simulink model "ball_balancing_omni3_multibody_lqi_rev1_r2024b"  (R2024b)
settings: Solver=VariableStepAuto  StartTime=0.0  StopTime=50  MaxStep=1e-3  MinStep=1e-6  RelTol=ballbotParams.simulation.relativeTolerance
PreLoadFcn:
  | if ~exist('ballbotParams','var'), ballbotParams = ballbotRev1Parameters; end
InitFcn:
  | if ~exist('ballbotParams','var') || ~isfield(ballbotParams,'parameterSource') || ballbotParams.parameterSource ~= "ballbotRev1Parameters" || ~isfield(ballbotParams,'controller') || ~isfield(ballbotParams,'estimator') || ~isfield(ballbotParams.controller,'torqueDrive') || ~isfield(ballbotParams.controller.torqueDrive,'propulsionGain') || ~isfield(ballbotParams.estimator,'truthDelaySteps') || ~isfield(ballbotParams.controller.torqueLqi,'robustness'), ballbotParams = ballbotRev1Parameters; end
  | % ballbotRev1RuntimeApply: re-apply runtime solver/driver/plant settings on every sim start.
  | clear functions;
  | ballbotRev1SimConfig;
  | if exist('ballbotParams','var'), ballbotRev1PlantAugment(bdroot, ballbotParams); end
values from neighbouring files (symbols this model uses):
  N = 0    [ballbotRollingResistance.m]
  s = result.spec    [ballbotBenchmark.m]
undefined symbols (not defined in the file or in its folder): ballbotCustomFriction, ballbotEstimatorInitialState, ballbotEstimatorUpdate, ballbotEulerToQuaternion, ballbotImuFromJoint, ballbotLqiControllerUpdate, ballbotLqiFeedbackState, ballbotMdd3aGateDrive, ballbotParams, ballbotPoseFromJoint, ballbotRev1CommandProfile, ballbotRollingResistance, ballbotRoverInitialPosition, ballbotShaftFrictionTorque, ballbotTorqueDutyStep, ballbotTruthGate, ballbotWheelRateFromDisplacement, X, Y, Z
libraries: nesl_utility x54, sm_lib x28, fl_lib x21, ee_lib x6
(part 2 of 3)

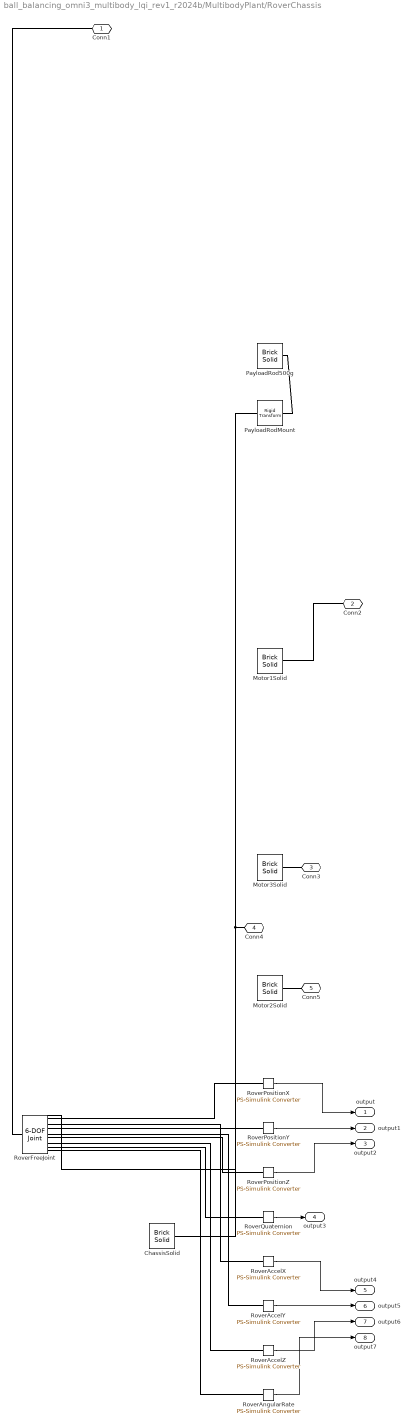
== system ball_balancing_omni3_multibody_lqi_rev1_r2024b/MultibodyPlant/RoverChassis ==
  ChassisSolid : sm_lib/Body Elements/Brick Solid  BrickDimensions=[0.12 0.12 ballbotParams.rover.chassisHeight]  BrickDimensionsUnits=m  ExportEntireGeometry=off  InertiaType=Custom  BasedOnType=Mass  Density=1000  DensityUnits=kg/m^3  Mass=ballbotParams.rover.bodyMass  MassUnits=kg  CenterOfMass=[0 0 ballbotParams.rover.bodyComAboveBall - ballbotParams.rover.centerAboveBall]  CenterOfMassUnits=m  MomentsOfInertia=ballbotParams.rover.bodyInertia.'  MomentsOfInertiaUnits=kg*m^2  ProductsOfInertia=[0 0 0]  ProductsOfInertiaUnits=kg*m^2  GraphicType=FromGeometry  MarkerShape=Sphere  MarkerSize=10  GraphicVisPropType=SimpleVisualProperties  GraphicDiffuseColor=[0.85 0.25 0.10 1.0]  GraphicOpacity=1  GraphicSpecularColor=[0.5 0.5 0.5 1.0]  GraphicAmbientColor=[0.15 0.15 0.15 1.0]  GraphicEmissiveColor=[0.0 0.0 0.0 1.0]  GraphicShininess=75  DoExposeReferenceFrame=on  SerializedFrames=<Frames/>
  Motor1Solid : sm_lib/Body Elements/Brick Solid  BrickDimensions=ballbotParams.motor.dimensions  BrickDimensionsUnits=m  ExportEntireGeometry=off  InertiaType=CalculateFromGeometry  BasedOnType=Mass  Density=1000  DensityUnits=kg/m^3  Mass=ballbotParams.motor.mass  MassUnits=kg  CenterOfMass=[0 0 0]  CenterOfMassUnits=m  MomentsOfInertia=[1 1 1]  MomentsOfInertiaUnits=kg*m^2  ProductsOfInertia=[0 0 0]  ProductsOfInertiaUnits=kg*m^2  GraphicType=FromGeometry  MarkerShape=Sphere  MarkerSize=10  GraphicVisPropType=SimpleVisualProperties  GraphicDiffuseColor=[0.25 0.25 0.25 1.0]  GraphicOpacity=1  GraphicSpecularColor=[0.5 0.5 0.5 1.0]  GraphicAmbientColor=[0.15 0.15 0.15 1.0]  GraphicEmissiveColor=[0.0 0.0 0.0 1.0]  GraphicShininess=75  DoExposeReferenceFrame=on  SerializedFrames=<Frames/>
  Motor2Solid : sm_lib/Body Elements/Brick Solid  BrickDimensions=ballbotParams.motor.dimensions  BrickDimensionsUnits=m  ExportEntireGeometry=off  InertiaType=CalculateFromGeometry  BasedOnType=Mass  Density=1000  DensityUnits=kg/m^3  Mass=ballbotParams.motor.mass  MassUnits=kg  CenterOfMass=[0 0 0]  CenterOfMassUnits=m  MomentsOfInertia=[1 1 1]  MomentsOfInertiaUnits=kg*m^2  ProductsOfInertia=[0 0 0]  ProductsOfInertiaUnits=kg*m^2  GraphicType=FromGeometry  MarkerShape=Sphere  MarkerSize=10  GraphicVisPropType=SimpleVisualProperties  GraphicDiffuseColor=[0.5 0.5 0.5]  GraphicOpacity=1  GraphicSpecularColor=[0.5 0.5 0.5 1.0]  GraphicAmbientColor=[0.15 0.15 0.15 1.0]  GraphicEmissiveColor=[0.0 0.0 0.0 1.0]  GraphicShininess=75  DoExposeReferenceFrame=on  SerializedFrames=<Frames/>
  Motor3Solid : sm_lib/Body Elements/Brick Solid  BrickDimensions=ballbotParams.motor.dimensions  BrickDimensionsUnits=m  ExportEntireGeometry=off  InertiaType=CalculateFromGeometry  BasedOnType=Mass  Density=1000  DensityUnits=kg/m^3  Mass=ballbotParams.motor.mass  MassUnits=kg  CenterOfMass=[0 0 0]  CenterOfMassUnits=m  MomentsOfInertia=[1 1 1]  MomentsOfInertiaUnits=kg*m^2  ProductsOfInertia=[0 0 0]  ProductsOfInertiaUnits=kg*m^2  GraphicType=FromGeometry  MarkerShape=Sphere  MarkerSize=10  GraphicVisPropType=SimpleVisualProperties  GraphicDiffuseColor=[0.5 0.5 0.5]  GraphicOpacity=1  GraphicSpecularColor=[0.5 0.5 0.5 1.0]  GraphicAmbientColor=[0.15 0.15 0.15 1.0]  GraphicEmissiveColor=[0.0 0.0 0.0 1.0]  GraphicShininess=75  DoExposeReferenceFrame=on  SerializedFrames=<Frames/>
  PayloadRod500g : sm_lib/Body Elements/Brick Solid  BrickDimensions=[ballbotParams.fullplant.payload.width ballbotParams.fullplant.payload.width ballbotParams.fullplant.payload.length]  BrickDimensionsUnits=m  ExportEntireGeometry=off  InertiaType=CalculateFromGeometry  BasedOnType=Density  Density=1000  DensityUnits=kg/m^3  Mass=ballbotParams.fullplant.payload.mass  MassUnits=kg  CenterOfMass=[0 0 0]  CenterOfMassUnits=m  MomentsOfInertia=[1 1 1]  MomentsOfInertiaUnits=kg*m^2  ProductsOfInertia=[0 0 0]  ProductsOfInertiaUnits=kg*m^2  GraphicType=FromGeometry  MarkerShape=Sphere  MarkerSize=10  GraphicVisPropType=SimpleVisualProperties  GraphicDiffuseColor=[0.5 0.5 0.5]  GraphicOpacity=1  GraphicSpecularColor=[0.5 0.5 0.5 1.0]  GraphicAmbientColor=[0.15 0.15 0.15 1.0]  GraphicEmissiveColor=[0.0 0.0 0.0 1.0]  GraphicShininess=75  DoExposeReferenceFrame=on  SerializedFrames=<Frames/>
  PayloadRodMount : sm_lib/Frames and Transforms/Rigid Transform  RotationMethod=None  FollAlignAxisA=+X  BaseAlignAxisA=+Y  FollAlignAxisB=+Y  BaseAlignAxisB=+Z  RotationStandardAxis=+Z  RotationAngle=0  RotationAngleUnits=deg  RotationArbitraryAxis=[0 0 1]  RotationSequenceAxes=FollowerAxes  RotationSequence=XYX  RotationSequenceAngles=[0 0 0]  RotationSequenceAnglesUnits=deg  RotationMatrix=[1 0 0;0 1 0;0 0 1]  Quaternion=[1 0 0 0]  TranslationMethod=Cartesian  TranslationCartesianOffset=[0 0 0.165]  TranslationCartesianOffsetUnits=m  TranslationStandardAxis=+Z  TranslationStandardOffset=0  TranslationStandardOffsetUnits=m  TranslationROffset=0  TranslationROffsetUnits=m  TranslationThetaOffset=0  TranslationThetaOffsetUnits=deg  TranslationZOffset=0  TranslationZOffsetUnits=m
  RoverAccelX : nesl_utility/PS-Simulink Converter  PhysicalDomain=network_engine_domain  SubClassName=ps_output  LeftPortType=input  RightPortType=output  PseudoPeriodic=off  Frequencies=[]  VectorFormat=inherit  Unit=m/s^2  AffineConversion=off
  RoverAccelY : nesl_utility/PS-Simulink Converter  PhysicalDomain=network_engine_domain  SubClassName=ps_output  LeftPortType=input  RightPortType=output  PseudoPeriodic=off  Frequencies=[]  VectorFormat=inherit  Unit=m/s^2  AffineConversion=off
  RoverAccelZ : nesl_utility/PS-Simulink Converter  PhysicalDomain=network_engine_domain  SubClassName=ps_output  LeftPortType=input  RightPortType=output  PseudoPeriodic=off  Frequencies=[]  VectorFormat=inherit  Unit=m/s^2  AffineConversion=off
  RoverAngularRate : nesl_utility/PS-Simulink Converter  PhysicalDomain=network_engine_domain  SubClassName=ps_output  LeftPortType=input  RightPortType=output  PseudoPeriodic=off  Frequencies=[]  VectorFormat=inherit  Unit=rad/s  AffineConversion=off
  RoverFreeJoint : sm_lib/Joints/6-DOF Joint  JointMode=Normal  CompositeWrenchDir=FollowerOnBase  CompositeWrenchFrame=BaseFrame  SenseConstraintForce=off  SenseConstraintTorque=off  SenseTotalForce=off  SenseTotalTorque=off  PxPositionTargetSpecify=on  PxPositionTargetPriority=High  PxPositionTargetValue=ballbotRoverInitialPosition(ballbotParams,1)  PxPositionTargetValueUnits=m  PxVelocityTargetSpecify=off  PxVelocityTargetPriority=High  PxVelocityTargetValue=0  PxVelocityTargetValueUnits=m/s  PxEquilibriumPosition=0  PxEquilibriumPositionUnits=m  PxSpringStiffness=0  PxSpringStiffnessUnits=N/m  PxDampingCoefficient=0  PxDampingCoefficientUnits=N/(m/s)  PxLowerLimitSpecify=off  PxLowerLimitBound=-1  PxLowerLimitBoundUnits=m  PxLowerLimitStiffness=1e6  PxLowerLimitStiffnessUnits=N/m  PxLowerLimitDamping=1e3  PxLowerLimitDampingUnits=N/(m/s)  PxLowerLimitTransitionRegionWidth=1e-4  PxLowerLimitTransitionRegionWidthUnits=m  PxUpperLimitSpecify=off  PxUpperLimitBound=1  PxUpperLimitBoundUnits=m  PxUpperLimitStiffness=1e6  PxUpperLimitStiffnessUnits=N/m  PxUpperLimitDamping=1e3  PxUpperLimitDampingUnits=N/(m/s)  PxUpperLimitTransitionRegionWidth=1e-4  PxUpperLimitTransitionRegionWidthUnits=m  PxTorqueActuationMode=NoTorque  PxMotionActuationMode=ComputedMotion  PxSensePosition=on  PxSenseVelocity=on  PxSenseAcceleration=on  PxSenseTorqueForce=off  PxSenseLowerLimitTorqueForce=off  PxSenseUpperLimitTorqueForce=off  PyPositionTargetSpecify=on  PyPositionTargetPriority=High  PyPositionTargetValue=ballbotRoverInitialPosition(ballbotParams,2)  PyPositionTargetValueUnits=m  PyVelocityTargetSpecify=off  PyVelocityTargetPriority=High  PyVelocityTargetValue=0  PyVelocityTargetValueUnits=m/s  PyEquilibriumPosition=0  PyEquilibriumPositionUnits=m  PySpringStiffness=0  PySpringStiffnessUnits=N/m  PyDampingCoefficient=0  PyDampingCoefficientUnits=N/(m/s)  PyLowerLimitSpecify=off  PyLowerLimitBound=-1  PyLowerLimitBoundUnits=m  PyLowerLimitStiffness=1e6  PyLowerLimitStiffnessUnits=N/m  PyLowerLimitDamping=1e3  PyLowerLimitDampingUnits=N/(m/s)  PyLowerLimitTransitionRegionWidth=1e-4  PyLowerLimitTransitionRegionWidthUnits=m  PyUpperLimitSpecify=off  PyUpperLimitBound=1  PyUpperLimitBoundUnits=m  PyUpperLimitStiffness=1e6  PyUpperLimitStiffnessUnits=N/m  PyUpperLimitDamping=1e3  PyUpperLimitDampingUnits=N/(m/s)  PyUpperLimitTransitionRegionWidth=1e-4  PyUpperLimitTransitionRegionWidthUnits=m  PyTorqueActuationMode=NoTorque  PyMotionActuationMode=ComputedMotion  PySensePosition=on  PySenseVelocity=on  PySenseAcceleration=on  PySenseTorqueForce=off  PySenseLowerLimitTorqueForce=off  PySenseUpperLimitTorqueForce=off  PzPositionTargetSpecify=on  PzPositionTargetPriority=High  PzPositionTargetValue=ballbotRoverInitialPosition(ballbotParams,3)  PzPositionTargetValueUnits=m  PzVelocityTargetSpecify=off  PzVelocityTargetPriority=High  PzVelocityTargetValue=0  PzVelocityTargetValueUnits=m/s  PzEquilibriumPosition=0  PzEquilibriumPositionUnits=m  PzSpringStiffness=0  PzSpringStiffnessUnits=N/m  PzDampingCoefficient=0  PzDampingCoefficientUnits=N/(m/s)  PzLowerLimitSpecify=off  PzLowerLimitBound=-1  PzLowerLimitBoundUnits=m  PzLowerLimitStiffness=1e6  PzLowerLimitStiffnessUnits=N/m  PzLowerLimitDamping=1e3  PzLowerLimitDampingUnits=N/(m/s)  PzLowerLimitTransitionRegionWidth=1e-4  PzLowerLimitTransitionRegionWidthUnits=m  PzUpperLimitSpecify=off  PzUpperLimitBound=1  PzUpperLimitBoundUnits=m  PzUpperLimitStiffness=1e6  PzUpperLimitStiffnessUnits=N/m  PzUpperLimitDamping=1e3  PzUpperLimitDampingUnits=N/(m/s)  PzUpperLimitTransitionRegionWidth=1e-4  PzUpperLimitTransitionRegionWidthUnits=m  PzTorqueActuationMode=NoTorque  PzMotionActuationMode=ComputedMotion  PzSensePosition=on  PzSenseVelocity=on  PzSenseAcceleration=on  PzSenseTorqueForce=off  PzSenseLowerLimitTorqueForce=off  PzSenseUpperLimitTorqueForce=off  SphPositionTargetSpecify=on  SphPositionTargetPriority=High  SphPositionTargetRotationMethod=Quaternion  SphPositionTargetFollAlignAxisA=+X  SphPositionTargetBaseAlignAxisA=+Y  SphPositionTargetFollAlignAxisB=+Y  SphPositionTargetBaseAlignAxisB=+Z  SphPositionTargetRotationStandardAxis=+Z  SphPositionTargetRotationAngle=0  SphPositionTargetRotationAngleUnits=deg  SphPositionTargetRotationArbitraryAxis=[0 0 1]  SphPositionTargetRotationSequenceAxes=FollowerAxes  SphPositionTargetRotationSequence=XYX  SphPositionTargetRotationSequenceAngles=[0 0 0]  SphPositionTargetRotationSequenceAnglesUnits=deg  SphPositionTargetRotationMatrix=[1 0 0;0 1 0;0 0 1]  SphPositionTargetQuaternion=ballbotEulerToQuaternion(ballbotParams.rover.initialEulerWorld)  SphVelocityTargetSpecify=off  SphVelocityTargetPriority=High  SphVelocityTargetValue=[0 0 0]  SphVelocityTargetValueUnits=deg/s  SphVelocityTargetInFollowerFrame=on  SphEqPosRotationMethod=None  SphEqPosFollAlignAxisA=+X  SphEqPosBaseAlignAxisA=+Y  SphEqPosFollAlignAxisB=+Y  SphEqPosBaseAlignAxisB=+Z  SphEqPosRotationStandardAxis=+Z  SphEqPosRotationAngle=0  SphEqPosRotationAngleUnits=deg  SphEqPosRotationArbitraryAxis=[0 0 1]  SphEqPosRotationSequenceAxes=FollowerAxes  SphEqPosRotationSequence=XYX  SphEqPosRotationSequenceAngles=[0 0 0]  SphEqPosRotationSequenceAnglesUnits=deg  SphEqPosRotationMatrix=[1 0 0;0 1 0;0 0 1]  SphEqPosQuaternion=[1 0 0 0]  SphSpringStiffness=0  SphSpringStiffnessUnits=N*m/deg  SphDampingCoefficient=0  SphDampingCoefficientUnits=N*m/(deg/s)  SphLowerLimitSpecify=off  SphLowerLimitBound=15  SphLowerLimitBoundUnits=deg  SphLowerLimitStiffness=1e4  SphLowerLimitStiffnessUnits=N*m/deg  SphLowerLimitDamping=10  SphLowerLimitDampingUnits=N*m/(deg/s)  SphLowerLimitTransitionRegionWidth=0.1  SphLowerLimitTransitionRegionWidthUnits=deg  SphUpperLimitSpecify=off  SphUpperLimitBound=45  SphUpperLimitBoundUnits=deg  SphUpperLimitStiffness=1e4  SphUpperLimitStiffnessUnits=N*m/deg  SphUpperLimitDamping=10  SphUpperLimitDampingUnits=N*m/(deg/s)  SphUpperLimitTransitionRegionWidth=0.1  SphUpperLimitTransitionRegionWidthUnits=deg  SphTorqueActuationMode=NoTorque  SphActuateTorqueX=off  SphActuateTorqueY=off  SphActuateTorqueZ=off  SphActuateTorque=off  SphActuationFrame=BaseFrame  SphSensePosition=on  SphSenseVelocityX=off  SphSenseVelocityY=off  SphSenseVelocityZ=off  SphSenseVelocity=on  SphSenseAccelerationX=off  SphSenseAccelerationY=off  SphSenseAccelerationZ=off  SphSenseAcceleration=on  SphSenseLowerLimitTorqueMag=off  SphSenseUpperLimitTorqueMag=off  SphSensingFrame=BaseFrame
  RoverPositionX : nesl_utility/PS-Simulink Converter  PhysicalDomain=network_engine_domain  SubClassName=ps_output  LeftPortType=input  RightPortType=output  PseudoPeriodic=off  Frequencies=[]  VectorFormat=inherit  Unit=m  AffineConversion=off
  RoverPositionY : nesl_utility/PS-Simulink Converter  PhysicalDomain=network_engine_domain  SubClassName=ps_output  LeftPortType=input  RightPortType=output  PseudoPeriodic=off  Frequencies=[]  VectorFormat=inherit  Unit=m  AffineConversion=off
  RoverPositionZ : nesl_utility/PS-Simulink Converter  PhysicalDomain=network_engine_domain  SubClassName=ps_output  LeftPortType=input  RightPortType=output  PseudoPeriodic=off  Frequencies=[]  VectorFormat=inherit  Unit=m  AffineConversion=off
  RoverQuaternion : nesl_utility/PS-Simulink Converter  PhysicalDomain=network_engine_domain  SubClassName=ps_output  LeftPortType=input  RightPortType=output  PseudoPeriodic=off  Frequencies=[]  VectorFormat=inherit  Unit=1  AffineConversion=off
  Conn1 : PMIOPort  Side=Left
  Conn2 : PMIOPort  Port=2  Side=Right
  Conn3 : PMIOPort  Port=3  Side=Right
  Conn4 : PMIOPort  Port=4  Side=Right
  Conn5 : PMIOPort  Port=5  Side=Right
  output : Outport
  output1 : Outport  Port=2
  output2 : Outport  Port=3
  output3 : Outport  Port=4
  output4 : Outport  Port=5
  output5 : Outport  Port=6
  output6 : Outport  Port=7
  output7 : Outport  Port=8
  wires:
  RoverAccelX/1 -> output4/1
  RoverPositionY/1 -> output1/1
  RoverAngularRate/1 -> output7/1
  RoverPositionX/1 -> output/1
  RoverAccelY/1 -> output5/1
  RoverPositionZ/1 -> output2/1
  RoverAccelZ/1 -> output6/1
  RoverQuaternion/1 -> output3/1
  connections:
  RoverFreeJoint/RConn4 -- RoverAccelX/LConn1
  RoverFreeJoint/RConn2 -- RoverPositionX/LConn1
  RoverFreeJoint/RConn11 -- RoverQuaternion/LConn1
  Conn3/RConn1 -- Motor3Solid/RConn1
  Conn2/RConn1 -- Motor1Solid/RConn1
  PayloadRodMount/RConn1 -- PayloadRod500g/RConn1
  RoverFreeJoint/RConn8 -- RoverPositionZ/LConn1
  RoverFreeJoint/RConn7 -- RoverAccelY/LConn1
  RoverFreeJoint/RConn10 -- RoverAccelZ/LConn1
  RoverFreeJoint/RConn12 -- RoverAngularRate/LConn1
  Conn5/RConn1 -- Motor2Solid/RConn1
  RoverFreeJoint/RConn5 -- RoverPositionY/LConn1
  Conn1/RConn1 -- RoverFreeJoint/LConn1
  Conn4/RConn1 -- RoverFreeJoint/RConn1 -- ChassisSolid/RConn1 -- PayloadRodMount/LConn1

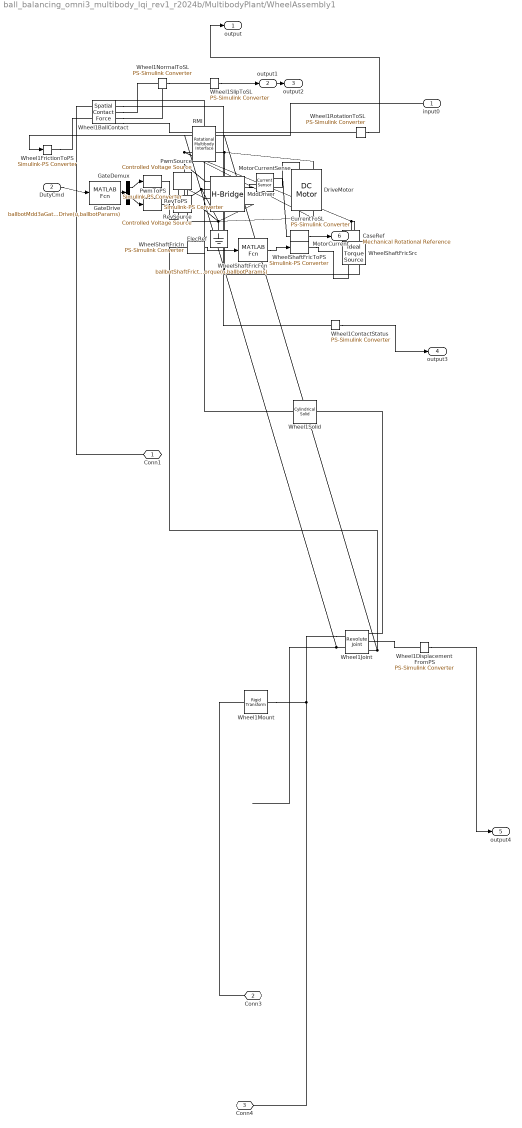
== system ball_balancing_omni3_multibody_lqi_rev1_r2024b/MultibodyPlant/WheelAssembly1 ==
  input0 : Inport
  DutyCmd : Inport  Port=2
  CaseRef : fl_lib/Mechanical/Rotational Elements/Mechanical Rotational Reference
  CurrentToSL : nesl_utility/PS-Simulink Converter  PhysicalDomain=network_engine_domain  SubClassName=ps_output  LeftPortType=input  RightPortType=output  PseudoPeriodic=off  Frequencies=[]  VectorFormat=inherit  Unit=A  AffineConversion=off
  DriveMotor : ee_lib/Electromechanical/Brushed Motors/DC Motor  field_option=ee.enum.field_option.pm  Rf=100 Ohm  Lf=1 H  Laf=0.15 H  If0=0 A  parameterization=ee.enum.dcparam_option.circuit_param  Ra=ballbotParams.motor.armatureResistance Ohm  La=ballbotParams.motor.armatureInductance H  emf_or_torque=ee.enum.emf_or_torque.ki  Kv=0.072e-3 V/rpm  Ki=ballbotParams.motor.torqueConstant N*m/A  T_stall=0.24e-3 N*m  w_max=19100 rpm  w_rated=15000 rpm  P_rated=0.08 W  V_rated=1.5 V  lam_param=ee.enum.lam_param.damping  i_noload=0 A  V_i_noload=1.5 V  J=ballbotParams.motor.equivalentInertia kg*m^2  lam=ballbotParams.motor.viscousFriction*ballbotParams.motor.viscousShare N*m*s/rad  speed0=0 rpm  alpha=3.93e-3 1/K  Tmeas=25 degC  thermal_mass=100 J/K  initial_temperature=25 degC
  ElecRef : fl_lib/Electrical/Electrical Elements/Electrical Reference
  GateDemux : Demux  Outputs=2
  GateDrive : MATLABFcn  MATLABFcn=ballbotMdd3aGateDrive(u,ballbotParams)  OutputDimensions=2
  MddDriver : ee_lib/Semiconductors & Converters/Converters/H-Bridge  pwm_or_av=ee.enum.pwm_or_av.averaged  discontinuous=ee.enum.current_profile.continuous  freewheeling_mode=ee.enum.converters.freewheeling_mode.one_switch_one_diode  Rload=10 Ohm  Lload=1e-5 H  F=ballbotParams.driver.pwmFrequency Hz  supply_ports=ee.enum.supply_ports.hidesupply  regenerative_braking_mode=ee.enum.converters.regenerative_braking_mode.always_enabled  Venable=ballbotParams.driver.enableThresholdVoltage V  Vmax=ballbotParams.driver.logicHighVoltage V  Vreverse=ballbotParams.driver.reverseThresholdVoltage V  Vbrake=ballbotParams.driver.brakeThresholdVoltage V  Vm=ballbotParams.driver.supplyVoltage V  Ron=ballbotParams.driver.bridgeOnResistance Ohm  Don=0.05 Ohm  Goff=1e-6 S  Tmeas=298.15 K  Ron2=0.1 Ohm  Don2=0.05 Ohm  Tmeas2=398.15 K  thermal_mass=100 J/K  initial_temperature=298.15 K
  MotorCurrentSense : fl_lib/Electrical/Electrical Sensors/Current Sensor
  PwmSource : fl_lib/Electrical/Electrical Sources/Controlled Voltage Source
  PwmToPS : nesl_utility/Simulink-PS Converter  PhysicalDomain=network_engine_domain  SubClassName=ps_input  LeftPortType=input  RightPortType=output  PseudoPeriodic=off  Frequencies=[]  NoiseDistribution=none  NoiseParameters=[]  Unit=1  AffineConversion=off  FilteringAndDerivatives=provide  SimscapeFilterOrder=1  InputFilterTimeConstant=0.001  UdotUserProvided=0
  RMI : fl_lib/Mechanical/Multibody Interfaces/Rotational Multibody Interface
  RevSource : fl_lib/Electrical/Electrical Sources/Controlled Voltage Source
  RevToPS : nesl_utility/Simulink-PS Converter  PhysicalDomain=network_engine_domain  SubClassName=ps_input  LeftPortType=input  RightPortType=output  PseudoPeriodic=off  Frequencies=[]  NoiseDistribution=none  NoiseParameters=[]  Unit=1  AffineConversion=off  FilteringAndDerivatives=provide  SimscapeFilterOrder=1  InputFilterTimeConstant=0.001  UdotUserProvided=0
  Wheel1BallContact : sm_lib/Forces and Torques/Spatial Contact Force  SenseSeparationDistance=off  NormalForceType=SmoothSpringDamper  NormalStiffness=ballbotParams.contact.wheelBall.normalStiffness  NormalStiffnessUnits=N/m  NormalDamping=ballbotParams.contact.wheelBall.normalDamping  NormalDampingUnits=N/(m/s)  NormalTransitionRegionWidth=ballbotParams.contact.wheelBall.relaxedTransitionWidth  NormalTransitionRegionWidthUnits=m  FrictionType=ProvidedByInput  CoefficientOfStaticFriction=ballbotParams.contact.wheelBall.staticFriction  CoefficientOfDynamicFriction=ballbotParams.contact.wheelBall.dynamicFriction  FrictionalCriticalVelocity=ballbotParams.contact.wheelBall.criticalVelocity  FrictionalCriticalVelocityUnits=m/s  SenseContactSignal=on  SensePenetrationDepth=off  SenseNormalVelocity=off  SenseTangentialVelocity=on  SensingForceTorqueDirection=BaseOnFollower  SensingForceTorqueResolutionFrame=ContactFrame  SenseNormalForce=off  SenseNormalForceMagnitude=on  SenseNormalTorque=off  SenseFrictionalForce=off  SenseFrictionalForceMagnitude=off  SenseFrictionalTorque=off  SenseTotalForce=off  SenseTotalTorque=off  SenseContactBaseRotation=off  SenseContactBaseTranslation=off  SenseContactFollowerRotation=on  SenseContactFollowerTranslation=off  ZeroCrossDetectContactStartAndEnd=on
  Wheel1ContactStatus : nesl_utility/PS-Simulink Converter  PhysicalDomain=network_engine_domain  SubClassName=ps_output  LeftPortType=input  RightPortType=output  PseudoPeriodic=off  Frequencies=[]  VectorFormat=inherit  Unit=1  AffineConversion=off
  Wheel1DisplacementFromPS : nesl_utility/PS-Simulink Converter  PhysicalDomain=network_engine_domain  SubClassName=ps_output  LeftPortType=input  RightPortType=output  PseudoPeriodic=off  Frequencies=[]  VectorFormat=inherit  Unit=rad  AffineConversion=off
  Wheel1FrictionToPS : nesl_utility/Simulink-PS Converter  PhysicalDomain=network_engine_domain  SubClassName=ps_input  LeftPortType=input  RightPortType=output  PseudoPeriodic=off  Frequencies=[]  NoiseDistribution=none  NoiseParameters=[]  Unit=N  AffineConversion=off  FilteringAndDerivatives=provide  SimscapeFilterOrder=1  InputFilterTimeConstant=0.001  UdotUserProvided=0
  Wheel1Joint : sm_lib/Joints/Revolute Joint  JointMode=Normal  CompositeWrenchDir=FollowerOnBase  CompositeWrenchFrame=BaseFrame  SenseConstraintForce=off  SenseConstraintTorque=off  SenseTotalForce=off  SenseTotalTorque=off  PositionTargetSpecify=off  PositionTargetPriority=High  PositionTargetValue=0  PositionTargetValueUnits=deg  VelocityTargetSpecify=off  VelocityTargetPriority=High  VelocityTargetValue=0  VelocityTargetValueUnits=deg/s  EquilibriumPosition=0  EquilibriumPositionUnits=deg  SpringStiffness=0  SpringStiffnessUnits=N*m/deg  DampingCoefficient=0  DampingCoefficientUnits=N*m/(deg/s)  LowerLimitSpecify=off  LowerLimitBound=-90  LowerLimitBoundUnits=deg  LowerLimitStiffness=1e4  LowerLimitStiffnessUnits=N*m/deg  LowerLimitDamping=10  LowerLimitDampingUnits=N*m/(deg/s)  LowerLimitTransitionRegionWidth=0.1  LowerLimitTransitionRegionWidthUnits=deg  UpperLimitSpecify=off  UpperLimitBound=90  UpperLimitBoundUnits=deg  UpperLimitStiffness=1e4  UpperLimitStiffnessUnits=N*m/deg  UpperLimitDamping=10  UpperLimitDampingUnits=N*m/(deg/s)  UpperLimitTransitionRegionWidth=0.1  UpperLimitTransitionRegionWidthUnits=deg  TorqueActuationMode=InputTorque  MotionActuationMode=ComputedMotion  SensePosition=on  SenseVelocity=on  SenseAcceleration=off  SenseTorqueForce=off  SenseLowerLimitTorqueForce=off  SenseUpperLimitTorqueForce=off
  Wheel1Mount : sm_lib/Frames and Transforms/Rigid Transform  RotationMethod=RotationMatrix  FollAlignAxisA=+X  BaseAlignAxisA=+Y  FollAlignAxisB=+Y  BaseAlignAxisB=+Z  RotationStandardAxis=+Z  RotationAngle=0  RotationAngleUnits=deg  RotationArbitraryAxis=[0 0 1]  RotationSequenceAxes=FollowerAxes  RotationSequence=XYX  RotationSequenceAngles=[0 0 0]  RotationSequenceAnglesUnits=deg  RotationMatrix=[ballbotParams.wheel.geometry.rollingBody(:,1),-ballbotParams.wheel.geometry.normalBody(:,1),ballbotParams.wheel.geometry.axleBody(:,1)]  Quaternion=[1 0 0 0]  TranslationMethod=Cartesian  TranslationCartesianOffset=ballbotParams.wheel.geometry.centerFromBody(:,1)'  TranslationCartesianOffsetUnits=m  TranslationStandardAxis=+Z  TranslationStandardOffset=0  TranslationStandardOffsetUnits=m  TranslationROffset=0  TranslationROffsetUnits=m  TranslationThetaOffset=0  TranslationThetaOffsetUnits=deg  TranslationZOffset=0  TranslationZOffsetUnits=m
  Wheel1NormalToSL : nesl_utility/PS-Simulink Converter  PhysicalDomain=network_engine_domain  SubClassName=ps_output  LeftPortType=input  RightPortType=output  PseudoPeriodic=off  Frequencies=[]  VectorFormat=inherit  Unit=N  AffineConversion=off
  Wheel1RotationToSL : nesl_utility/PS-Simulink Converter  PhysicalDomain=network_engine_domain  SubClassName=ps_output  LeftPortType=input  RightPortType=output  PseudoPeriodic=off  Frequencies=[]  VectorFormat=inherit  Unit=1  AffineConversion=off
  Wheel1SlipToSL : nesl_utility/PS-Simulink Converter  PhysicalDomain=network_engine_domain  SubClassName=ps_output  LeftPortType=input  RightPortType=output  PseudoPeriodic=off  Frequencies=[]  VectorFormat=inherit  Unit=m/s  AffineConversion=off
  Wheel1Solid : sm_lib/Body Elements/Cylindrical Solid  CylinderRadius=ballbotParams.wheel.radius  CylinderRadiusUnits=m  CylinderLength=ballbotParams.wheel.width  CylinderLengthUnits=m  ExportEntireGeometry=on  InertiaType=CalculateFromGeometry  BasedOnType=Mass  Density=1000  DensityUnits=kg/m^3  Mass=ballbotParams.wheel.mass  MassUnits=kg  CenterOfMass=[0 0 0]  CenterOfMassUnits=m  MomentsOfInertia=[1 1 1]  MomentsOfInertiaUnits=kg*m^2  ProductsOfInertia=[0 0 0]  ProductsOfInertiaUnits=kg*m^2  GraphicType=FromGeometry  MarkerShape=Sphere  MarkerSize=10  GraphicVisPropType=SimpleVisualProperties  GraphicDiffuseColor=[0.08 0.08 0.08 1.0]  GraphicOpacity=1  GraphicSpecularColor=[0.5 0.5 0.5 1.0]  GraphicAmbientColor=[0.15 0.15 0.15 1.0]  GraphicEmissiveColor=[0.0 0.0 0.0 1.0]  GraphicShininess=75  DoExposeReferenceFrame=on  SerializedFrames=<Frames/>
  WheelShaftFricFcn : MATLABFcn  MATLABFcn=ballbotShaftFrictionTorque(u,ballbotParams)
  WheelShaftFricIn : nesl_utility/PS-Simulink Converter  PhysicalDomain=network_engine_domain  SubClassName=ps_output  LeftPortType=input  RightPortType=output  PseudoPeriodic=off  Frequencies=[]  VectorFormat=inherit  Unit=rad/s  AffineConversion=off
  WheelShaftFricSrc : fl_lib/Mechanical/Mechanical Sources/Ideal Torque Source
  WheelShaftFricToPS : nesl_utility/Simulink-PS Converter  PhysicalDomain=network_engine_domain  SubClassName=ps_input  LeftPortType=input  RightPortType=output  PseudoPeriodic=off  Frequencies=[]  NoiseDistribution=none  NoiseParameters=[]  Unit=N*m  AffineConversion=off  FilteringAndDerivatives=provide  SimscapeFilterOrder=1  InputFilterTimeConstant=0.001  UdotUserProvided=0
  Conn1 : PMIOPort  Side=Left
  Conn3 : PMIOPort  Port=2  Side=Left
  Conn4 : PMIOPort  Port=3  Side=Left
  output : Outport
  output1 : Outport  Port=2
  output2 : Outport  Port=3
  output3 : Outport  Port=4
  output4 : Outport  Port=5
  MotorCurrent : Outport  Port=6
  wires:
  Wheel1RotationToSL/1 -> output/1
  Wheel1NormalToSL/1 -> output1/1
  Wheel1ContactStatus/1 -> output3/1
  input0/1 -> Wheel1FrictionToPS/1
  Wheel1DisplacementFromPS/1 -> output4/1
  Wheel1SlipToSL/1 -> output2/1
  DutyCmd/1 -> GateDrive/1
  GateDrive/1 -> GateDemux/1
  GateDemux/1 -> PwmToPS/1
  GateDemux/2 -> RevToPS/1
  CurrentToSL/1 -> MotorCurrent/1
  WheelShaftFricIn/1 -> WheelShaftFricFcn/1
  WheelShaftFricFcn/1 -> WheelShaftFricToPS/1
  connections:
  Wheel1BallContact/LConn1 -- Conn1/RConn1
  Wheel1BallContact/RConn3 -- Wheel1NormalToSL/LConn1
  Wheel1Joint/RConn1 -- Wheel1Solid/RConn1
  Wheel1BallContact/RConn4 -- Wheel1SlipToSL/LConn1
  Wheel1BallContact/RConn2 -- Wheel1ContactStatus/LConn1
  Wheel1FrictionToPS/RConn1 -- Wheel1BallContact/LConn2
  Wheel1Joint/LConn1 -- Conn4/RConn1 -- Wheel1Mount/RConn1
  Wheel1Joint/RConn2 -- Wheel1DisplacementFromPS/LConn1
  Wheel1Solid/LConn1 -- Wheel1BallContact/RConn1
  Wheel1BallContact/RConn5 -- Wheel1RotationToSL/LConn1
  Conn3/RConn1 -- Wheel1Mount/LConn1
  Wheel1Joint/LConn2 -- RMI/LConn1
  PwmToPS/RConn1 -- PwmSource/RConn1
  RevToPS/RConn1 -- RevSource/RConn1
  PwmSource/LConn1 -- MddDriver/LConn1
  RevSource/LConn1 -- MddDriver/LConn3
  RevSource/RConn2 -- MddDriver/LConn4 -- DriveMotor/RConn1 -- MddDriver/RConn2 -- ElecRef/LConn1 -- PwmSource/RConn2 -- MddDriver/LConn2
  MddDriver/RConn1 -- MotorCurrentSense/LConn1
  MotorCurrentSense/RConn2 -- DriveMotor/LConn1
  MotorCurrentSense/RConn1 -- CurrentToSL/LConn1
  RMI/RConn2 -- DriveMotor/LConn2 -- WheelShaftFricSrc/RConn2
  RMI/LConn2 -- DriveMotor/RConn2 -- CaseRef/LConn1 -- WheelShaftFricSrc/LConn1
  RMI/RConn1 -- Wheel1Joint/RConn3 -- WheelShaftFricIn/LConn1
  WheelShaftFricToPS/RConn1 -- WheelShaftFricSrc/RConn1

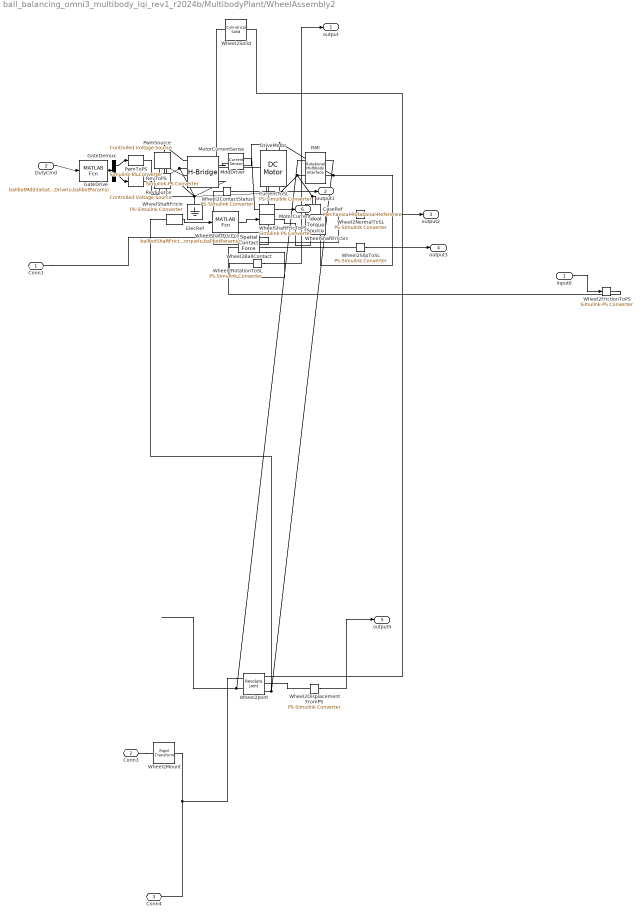
== system ball_balancing_omni3_multibody_lqi_rev1_r2024b/MultibodyPlant/WheelAssembly2 ==
  input0 : Inport
  DutyCmd : Inport  Port=2
  CaseRef : fl_lib/Mechanical/Rotational Elements/Mechanical Rotational Reference
  CurrentToSL : nesl_utility/PS-Simulink Converter  PhysicalDomain=network_engine_domain  SubClassName=ps_output  LeftPortType=input  RightPortType=output  PseudoPeriodic=off  Frequencies=[]  VectorFormat=inherit  Unit=A  AffineConversion=off
  DriveMotor : ee_lib/Electromechanical/Brushed Motors/DC Motor  field_option=ee.enum.field_option.pm  Rf=100 Ohm  Lf=1 H  Laf=0.15 H  If0=0 A  parameterization=ee.enum.dcparam_option.circuit_param  Ra=ballbotParams.motor.armatureResistance Ohm  La=ballbotParams.motor.armatureInductance H  emf_or_torque=ee.enum.emf_or_torque.ki  Kv=0.072e-3 V/rpm  Ki=ballbotParams.motor.torqueConstant N*m/A  T_stall=0.24e-3 N*m  w_max=19100 rpm  w_rated=15000 rpm  P_rated=0.08 W  V_rated=1.5 V  lam_param=ee.enum.lam_param.damping  i_noload=0 A  V_i_noload=1.5 V  J=ballbotParams.motor.equivalentInertia kg*m^2  lam=ballbotParams.motor.viscousFriction*ballbotParams.motor.viscousShare N*m*s/rad  speed0=0 rpm  alpha=3.93e-3 1/K  Tmeas=25 degC  thermal_mass=100 J/K  initial_temperature=25 degC
  ElecRef : fl_lib/Electrical/Electrical Elements/Electrical Reference
  GateDemux : Demux  Outputs=2
  GateDrive : MATLABFcn  MATLABFcn=ballbotMdd3aGateDrive(u,ballbotParams)  OutputDimensions=2
  MddDriver : ee_lib/Semiconductors & Converters/Converters/H-Bridge  pwm_or_av=ee.enum.pwm_or_av.averaged  discontinuous=ee.enum.current_profile.continuous  freewheeling_mode=ee.enum.converters.freewheeling_mode.one_switch_one_diode  Rload=10 Ohm  Lload=1e-5 H  F=ballbotParams.driver.pwmFrequency Hz  supply_ports=ee.enum.supply_ports.hidesupply  regenerative_braking_mode=ee.enum.converters.regenerative_braking_mode.always_enabled  Venable=ballbotParams.driver.enableThresholdVoltage V  Vmax=ballbotParams.driver.logicHighVoltage V  Vreverse=ballbotParams.driver.reverseThresholdVoltage V  Vbrake=ballbotParams.driver.brakeThresholdVoltage V  Vm=ballbotParams.driver.supplyVoltage V  Ron=ballbotParams.driver.bridgeOnResistance Ohm  Don=0.05 Ohm  Goff=1e-6 S  Tmeas=298.15 K  Ron2=0.1 Ohm  Don2=0.05 Ohm  Tmeas2=398.15 K  thermal_mass=100 J/K  initial_temperature=298.15 K
  MotorCurrentSense : fl_lib/Electrical/Electrical Sensors/Current Sensor
  PwmSource : fl_lib/Electrical/Electrical Sources/Controlled Voltage Source
  PwmToPS : nesl_utility/Simulink-PS Converter  PhysicalDomain=network_engine_domain  SubClassName=ps_input  LeftPortType=input  RightPortType=output  PseudoPeriodic=off  Frequencies=[]  NoiseDistribution=none  NoiseParameters=[]  Unit=1  AffineConversion=off  FilteringAndDerivatives=provide  SimscapeFilterOrder=1  InputFilterTimeConstant=0.001  UdotUserProvided=0
  RMI : fl_lib/Mechanical/Multibody Interfaces/Rotational Multibody Interface
  RevSource : fl_lib/Electrical/Electrical Sources/Controlled Voltage Source
  RevToPS : nesl_utility/Simulink-PS Converter  PhysicalDomain=network_engine_domain  SubClassName=ps_input  LeftPortType=input  RightPortType=output  PseudoPeriodic=off  Frequencies=[]  NoiseDistribution=none  NoiseParameters=[]  Unit=1  AffineConversion=off  FilteringAndDerivatives=provide  SimscapeFilterOrder=1  InputFilterTimeConstant=0.001  UdotUserProvided=0
  Wheel2BallContact : sm_lib/Forces and Torques/Spatial Contact Force  SenseSeparationDistance=off  NormalForceType=SmoothSpringDamper  NormalStiffness=ballbotParams.contact.wheelBall.normalStiffness  NormalStiffnessUnits=N/m  NormalDamping=ballbotParams.contact.wheelBall.normalDamping  NormalDampingUnits=N/(m/s)  NormalTransitionRegionWidth=ballbotParams.contact.wheelBall.relaxedTransitionWidth  NormalTransitionRegionWidthUnits=m  FrictionType=ProvidedByInput  CoefficientOfStaticFriction=ballbotParams.contact.wheelBall.staticFriction  CoefficientOfDynamicFriction=ballbotParams.contact.wheelBall.dynamicFriction  FrictionalCriticalVelocity=ballbotParams.contact.wheelBall.criticalVelocity  FrictionalCriticalVelocityUnits=m/s  SenseContactSignal=on  SensePenetrationDepth=off  SenseNormalVelocity=off  SenseTangentialVelocity=on  SensingForceTorqueDirection=BaseOnFollower  SensingForceTorqueResolutionFrame=ContactFrame  SenseNormalForce=off  SenseNormalForceMagnitude=on  SenseNormalTorque=off  SenseFrictionalForce=off  SenseFrictionalForceMagnitude=off  SenseFrictionalTorque=off  SenseTotalForce=off  SenseTotalTorque=off  SenseContactBaseRotation=off  SenseContactBaseTranslation=off  SenseContactFollowerRotation=on  SenseContactFollowerTranslation=off  ZeroCrossDetectContactStartAndEnd=on
  Wheel2ContactStatus : nesl_utility/PS-Simulink Converter  PhysicalDomain=network_engine_domain  SubClassName=ps_output  LeftPortType=input  RightPortType=output  PseudoPeriodic=off  Frequencies=[]  VectorFormat=inherit  Unit=1  AffineConversion=off
  Wheel2DisplacementFromPS : nesl_utility/PS-Simulink Converter  PhysicalDomain=network_engine_domain  SubClassName=ps_output  LeftPortType=input  RightPortType=output  PseudoPeriodic=off  Frequencies=[]  VectorFormat=inherit  Unit=rad  AffineConversion=off
  Wheel2FrictionToPS : nesl_utility/Simulink-PS Converter  PhysicalDomain=network_engine_domain  SubClassName=ps_input  LeftPortType=input  RightPortType=output  PseudoPeriodic=off  Frequencies=[]  NoiseDistribution=none  NoiseParameters=[]  Unit=N  AffineConversion=off  FilteringAndDerivatives=provide  SimscapeFilterOrder=1  InputFilterTimeConstant=0.001  UdotUserProvided=0
  Wheel2Joint : sm_lib/Joints/Revolute Joint  JointMode=Normal  CompositeWrenchDir=FollowerOnBase  CompositeWrenchFrame=BaseFrame  SenseConstraintForce=off  SenseConstraintTorque=off  SenseTotalForce=off  SenseTotalTorque=off  PositionTargetSpecify=off  PositionTargetPriority=High  PositionTargetValue=0  PositionTargetValueUnits=deg  VelocityTargetSpecify=off  VelocityTargetPriority=High  VelocityTargetValue=0  VelocityTargetValueUnits=deg/s  EquilibriumPosition=0  EquilibriumPositionUnits=deg  SpringStiffness=0  SpringStiffnessUnits=N*m/deg  DampingCoefficient=0  DampingCoefficientUnits=N*m/(deg/s)  LowerLimitSpecify=off  LowerLimitBound=-90  LowerLimitBoundUnits=deg  LowerLimitStiffness=1e4  LowerLimitStiffnessUnits=N*m/deg  LowerLimitDamping=10  LowerLimitDampingUnits=N*m/(deg/s)  LowerLimitTransitionRegionWidth=0.1  LowerLimitTransitionRegionWidthUnits=deg  UpperLimitSpecify=off  UpperLimitBound=90  UpperLimitBoundUnits=deg  UpperLimitStiffness=1e4  UpperLimitStiffnessUnits=N*m/deg  UpperLimitDamping=10  UpperLimitDampingUnits=N*m/(deg/s)  UpperLimitTransitionRegionWidth=0.1  UpperLimitTransitionRegionWidthUnits=deg  TorqueActuationMode=InputTorque  MotionActuationMode=ComputedMotion  SensePosition=on  SenseVelocity=on  SenseAcceleration=off  SenseTorqueForce=off  SenseLowerLimitTorqueForce=off  SenseUpperLimitTorqueForce=off
  Wheel2Mount : sm_lib/Frames and Transforms/Rigid Transform  RotationMethod=RotationMatrix  FollAlignAxisA=+X  BaseAlignAxisA=+Y  FollAlignAxisB=+Y  BaseAlignAxisB=+Z  RotationStandardAxis=+Z  RotationAngle=0  RotationAngleUnits=deg  RotationArbitraryAxis=[0 0 1]  RotationSequenceAxes=FollowerAxes  RotationSequence=XYX  RotationSequenceAngles=[0 0 0]  RotationSequenceAnglesUnits=deg  RotationMatrix=[ballbotParams.wheel.geometry.rollingBody(:,2),-ballbotParams.wheel.geometry.normalBody(:,2),ballbotParams.wheel.geometry.axleBody(:,2)]  Quaternion=[1 0 0 0]  TranslationMethod=Cartesian  TranslationCartesianOffset=ballbotParams.wheel.geometry.centerFromBody(:,2)'  TranslationCartesianOffsetUnits=m  TranslationStandardAxis=+Z  TranslationStandardOffset=0  TranslationStandardOffsetUnits=m  TranslationROffset=0  TranslationROffsetUnits=m  TranslationThetaOffset=0  TranslationThetaOffsetUnits=deg  TranslationZOffset=0  TranslationZOffsetUnits=m
  Wheel2NormalToSL : nesl_utility/PS-Simulink Converter  PhysicalDomain=network_engine_domain  SubClassName=ps_output  LeftPortType=input  RightPortType=output  PseudoPeriodic=off  Frequencies=[]  VectorFormat=inherit  Unit=N  AffineConversion=off
  Wheel2RotationToSL : nesl_utility/PS-Simulink Converter  PhysicalDomain=network_engine_domain  SubClassName=ps_output  LeftPortType=input  RightPortType=output  PseudoPeriodic=off  Frequencies=[]  VectorFormat=inherit  Unit=1  AffineConversion=off
  Wheel2SlipToSL : nesl_utility/PS-Simulink Converter  PhysicalDomain=network_engine_domain  SubClassName=ps_output  LeftPortType=input  RightPortType=output  PseudoPeriodic=off  Frequencies=[]  VectorFormat=inherit  Unit=m/s  AffineConversion=off
  Wheel2Solid : sm_lib/Body Elements/Cylindrical Solid  CylinderRadius=ballbotParams.wheel.radius  CylinderRadiusUnits=m  CylinderLength=ballbotParams.wheel.width  CylinderLengthUnits=m  ExportEntireGeometry=on  InertiaType=CalculateFromGeometry  BasedOnType=Mass  Density=1000  DensityUnits=kg/m^3  Mass=ballbotParams.wheel.mass  MassUnits=kg  CenterOfMass=[0 0 0]  CenterOfMassUnits=m  MomentsOfInertia=[1 1 1]  MomentsOfInertiaUnits=kg*m^2  ProductsOfInertia=[0 0 0]  ProductsOfInertiaUnits=kg*m^2  GraphicType=FromGeometry  MarkerShape=Sphere  MarkerSize=10  GraphicVisPropType=SimpleVisualProperties  GraphicDiffuseColor=[0.5 0.5 0.5]  GraphicOpacity=1  GraphicSpecularColor=[0.5 0.5 0.5 1.0]  GraphicAmbientColor=[0.15 0.15 0.15 1.0]  GraphicEmissiveColor=[0.0 0.0 0.0 1.0]  GraphicShininess=75  DoExposeReferenceFrame=on  SerializedFrames=<Frames/>
  WheelShaftFricFcn : MATLABFcn  MATLABFcn=ballbotShaftFrictionTorque(u,ballbotParams)
  WheelShaftFricIn : nesl_utility/PS-Simulink Converter  PhysicalDomain=network_engine_domain  SubClassName=ps_output  LeftPortType=input  RightPortType=output  PseudoPeriodic=off  Frequencies=[]  VectorFormat=inherit  Unit=rad/s  AffineConversion=off
  WheelShaftFricSrc : fl_lib/Mechanical/Mechanical Sources/Ideal Torque Source
  WheelShaftFricToPS : nesl_utility/Simulink-PS Converter  PhysicalDomain=network_engine_domain  SubClassName=ps_input  LeftPortType=input  RightPortType=output  PseudoPeriodic=off  Frequencies=[]  NoiseDistribution=none  NoiseParameters=[]  Unit=N*m  AffineConversion=off  FilteringAndDerivatives=provide  SimscapeFilterOrder=1  InputFilterTimeConstant=0.001  UdotUserProvided=0
  Conn1 : PMIOPort  Side=Left
  Conn3 : PMIOPort  Port=2  Side=Left
  Conn4 : PMIOPort  Port=3  Side=Left
  output : Outport
  output1 : Outport  Port=2
  output2 : Outport  Port=3
  output3 : Outport  Port=4
  output4 : Outport  Port=5
  MotorCurrent : Outport  Port=6
  wires:
  Wheel2RotationToSL/1 -> output/1
  input0/1 -> Wheel2FrictionToPS/1
  Wheel2NormalToSL/1 -> output2/1
  Wheel2SlipToSL/1 -> output3/1
  Wheel2DisplacementFromPS/1 -> output4/1
  Wheel2ContactStatus/1 -> output1/1
  DutyCmd/1 -> GateDrive/1
  GateDrive/1 -> GateDemux/1
  GateDemux/1 -> PwmToPS/1
  GateDemux/2 -> RevToPS/1
  CurrentToSL/1 -> MotorCurrent/1
  WheelShaftFricIn/1 -> WheelShaftFricFcn/1
  WheelShaftFricFcn/1 -> WheelShaftFricToPS/1
  connections:
  Wheel2BallContact/RConn5 -- Wheel2RotationToSL/LConn1
  Wheel2Joint/LConn1 -- Conn4/RConn1 -- Wheel2Mount/RConn1
  Wheel2Joint/RConn1 -- Wheel2Solid/RConn1
  Wheel2BallContact/RConn3 -- Wheel2NormalToSL/LConn1
  Wheel2BallContact/RConn2 -- Wheel2ContactStatus/LConn1
  Wheel2FrictionToPS/RConn1 -- Wheel2BallContact/LConn2
  Wheel2Joint/RConn2 -- Wheel2DisplacementFromPS/LConn1
  Wheel2Solid/LConn1 -- Wheel2BallContact/RConn1
  Wheel2BallContact/RConn4 -- Wheel2SlipToSL/LConn1
  Conn3/RConn1 -- Wheel2Mount/LConn1
  Wheel2Joint/LConn2 -- RMI/LConn1
  Conn1/RConn1 -- Wheel2BallContact/LConn1
  PwmToPS/RConn1 -- PwmSource/RConn1
  RevToPS/RConn1 -- RevSource/RConn1
  PwmSource/LConn1 -- MddDriver/LConn1
  RevSource/LConn1 -- MddDriver/LConn3
  RevSource/RConn2 -- MddDriver/LConn4 -- DriveMotor/RConn1 -- MddDriver/RConn2 -- ElecRef/LConn1 -- PwmSource/RConn2 -- MddDriver/LConn2
  MddDriver/RConn1 -- MotorCurrentSense/LConn1
  MotorCurrentSense/RConn2 -- DriveMotor/LConn1
  MotorCurrentSense/RConn1 -- CurrentToSL/LConn1
  RMI/RConn2 -- DriveMotor/LConn2 -- WheelShaftFricSrc/RConn2
  RMI/LConn2 -- DriveMotor/RConn2 -- CaseRef/LConn1 -- WheelShaftFricSrc/LConn1
  RMI/RConn1 -- Wheel2Joint/RConn3 -- WheelShaftFricIn/LConn1
  WheelShaftFricToPS/RConn1 -- WheelShaftFricSrc/RConn1
